simulink model "simulator_model_G"  (R2023b)
settings: Solver=ode4  StartTime=0.0  StopTime=10  FixedStep=0.01  RelTol=1e-3
values from neighbouring files (symbols this model uses):
  Fv = 0.04    [main.m]
  g = Simulink.Parameter(9.81)    [main.m]
  I1 = Simulink.Parameter( (1/12)*m1.Value*(l1.Value^2) )    [main.m]
  I2 = Simulink.Parameter( (1/12)*m2.Value*(l2.Value^2) )    [main.m]
  l1 = Simulink.Parameter(1)    [main.m]    (also in plot_robot.m = inputs(3); plot_robot_3links.m = inputs(4))
  l2 = Simulink.Parameter(1)    [main.m]    (also in plot_robot.m = inputs(4); plot_robot_3links.m = inputs(5))
  lc1 = Simulink.Parameter(l1.Value/2)    [main.m]
  lc2 = Simulink.Parameter(l2.Value/2)    [main.m]
  m1 = Simulink.Parameter(0.5)    [main.m]
  m2 = Simulink.Parameter(0.2)    [main.m]
settings Model: Creator=Gabriel  LastModifiedBy=Bruno

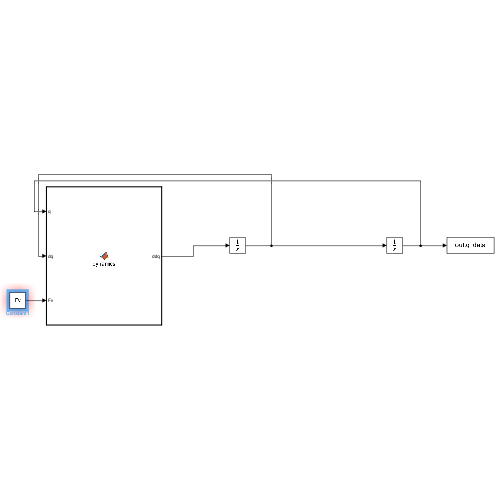
[thumbnail: Simulink's stored preview of the top-level diagram]
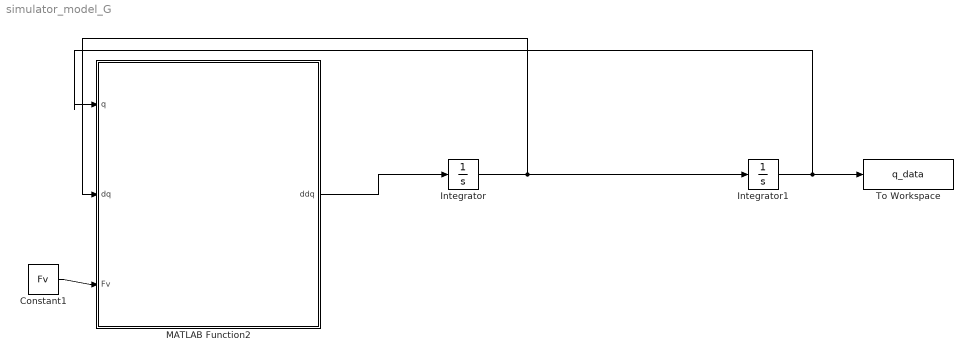
== system simulator_model_G ==
  Constant1 : Constant  Value=Fv
  Integrator : Integrator  InitialCondition=[0;0]
  Integrator1 : Integrator  InitialCondition=[pi/2;pi/4]
  MATLAB Function2 : MATLAB Function  TreatAsAtomicUnit=on
  To Workspace : ToWorkspace  VariableName=q_data  SampleTime=-1
      settings: Save2DSignal=2-D array (concatenate along first dimension)
  wires:
  Integrator/1 -> MATLAB Function2/2(dq), Integrator1/1
  Integrator1/1 -> To Workspace/1, MATLAB Function2/1(q)
  MATLAB Function2/1(ddq) -> Integrator/1
  Constant1/1 -> MATLAB Function2/3(Fv)

== matlab function simulator_model_G/MATLAB Function2 ==
  data: q input; ddq output; dq input; Fv input; m1 parameter; m2 parameter; l1 parameter; l2 parameter; lc1 parameter; lc2 parameter; I1 parameter; I2 parameter; g parameter
function ddq = dynamics(q,dq,Fv,m1, m2, l1, l2, lc1, lc2, I1, I2, g)
M = mass_matrix(q(1),q(2),m1,m2,l1,l2,lc1,lc2,I1,I2);
C = coriolis_matrix(q(1),q(2),dq(1),dq(2),m1,m2,l1,l2,lc1,lc2);
G = gravity_vector(q(1),q(2),m1,m2,l1,l2,lc1,lc2,g);
tau = G;
ddq = M \ (tau - C*dq - G - Fv * dq);
